simulink model "skarab_hmc_test"  (R2018a)
settings: Solver=VariableStepDiscrete  StartTime=0.0  StopTime=256.0  RelTol=1e-3
libraries: xbsIndex_r4 x424, xps_library x2
(part 1 of 4)
settings Model: Creator=omer  LastModifiedBy=hpw1
settings DataIOCC: LimitDataPoints=on  SaveFormat=Array
settings OptimizationCC: DefaultParameterBehavior=Inlined  ExpressionDepthLimit=2147483647  LifeSpan=inf
settings DebuggingCC: UnderspecifiedInitializationDetection=Classic  MergeDetectMultiDrivingBlocksExec=none  SolverPrmCheckMsg=warning  AllowSymbolicDim=off  StateNameClashWarn=warning  LibraryContextMissingDiagnostic=warning  SFUnexpectedBacktrackingDiag=warning  SFNoUnconditionalDefaultTransitionDiag=warning  SFExecutionAtInitializationDiag=none
settings HardwareCC: ProdBitPerPointer=32  ProdBitPerSizeT=32  ProdBitPerPtrDiffT=32  ProdLargestAtomicFloat=None  ProdIntDivRoundTo=Undefined  ProdEndianess=Unspecified  ProdWordSize=32  ProdHWDeviceType=32-bit Generic
settings ModelReferenceCC: PropagateSignalLabelsOutOfModel=off
settings CodeAppCC: StateflowObjectComments=on
settings GRTTargetCC: TargetLangStandard=C89/C90 (ANSI)  GeneratePreprocessorConditionals=Disable all
settings ConfigComp: CovMetricSettings=dw  CovHtmlReporting=on  CovSaveCumulativeToWorkspaceVar=on  CovSaveSingleToWorkspaceVar=on  CovExternalEMLEnable=off

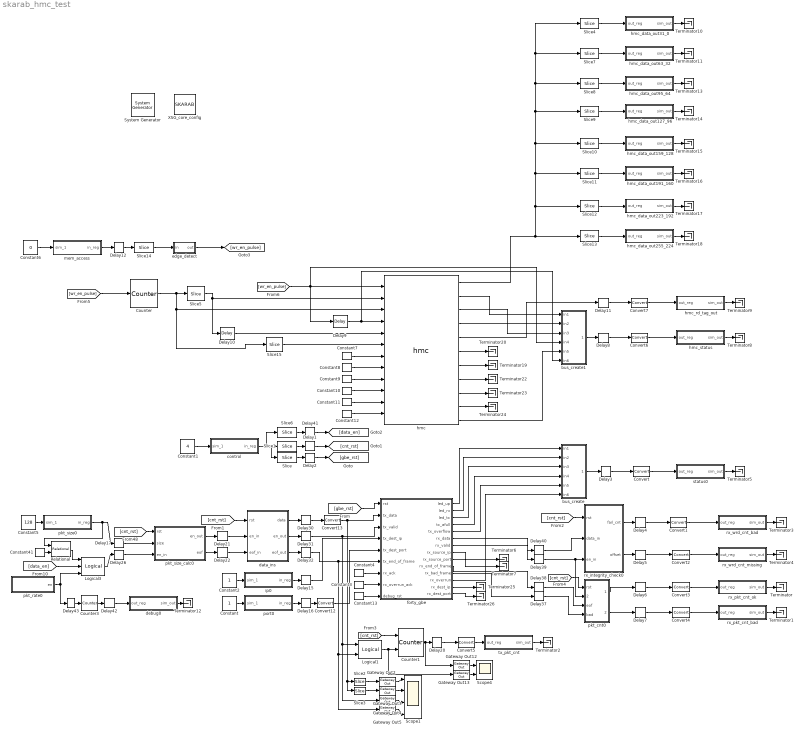
== system skarab_hmc_test ==
  " System Generator" : xbsIndex_r4/ System Generator  Tag=genX  xilinxfamily=virtex7  part=xc7vx690t  speed=-2  package=ffg1927  synthesis_tool=XST  clock_wrapper=Clock Enables  directory=/home/aisaacson/work/git_work/ska_sa/projects/mlib_devel/jasper_library/test_models/skarab_hmc_test/sysgen  proj_type=Vivado  Synth_file=Vivado Synthesis Defaults  Impl_file=Vivado Implementation Defaults  testbench=off  simulink_period=1  sysclk_period=4.4444  dcm_input_clock_period=10  incr_netlist=off  trim_vbits=Everywhere in SubSystem  dbl_ovrd=According to Block Masks  core_generation=According to Block Masks  run_coregen=off  deprecated_control=off  eval_field=0  block_type=sysgen
  Constant : Constant
  Constant1 : Constant  Value=4
  Constant10 : xbsIndex_r4/Constant  const=0  gui_display_data_type=Boolean  arith_type=Boolean  n_bits=16  bin_pt=14  preci_type=Single  exp_width=8  frac_width=24  explicit_period=on  period=1  equ=P=C  opselect=C  inp2=PCIN>>17  opr=+  inp1=P  carry=CIN  dbl_ovrd=off  block_type=constant
      settings: block_version=11.4
  Constant11 : xbsIndex_r4/Constant  const=0  gui_display_data_type=Fixed-point  arith_type=Unsigned  n_bits=27  bin_pt=0  preci_type=Single  exp_width=8  frac_width=24  explicit_period=on  period=1  equ=P=C  opselect=C  inp2=PCIN>>17  opr=+  inp1=P  carry=CIN  dbl_ovrd=off  block_type=constant
      settings: block_version=11.4
  Constant12 : xbsIndex_r4/Constant  const=0  gui_display_data_type=Fixed-point  arith_type=Signed (2's comp)  n_bits=9  bin_pt=0  preci_type=Single  exp_width=8  frac_width=24  explicit_period=on  period=1  equ=P=C  opselect=C  inp2=PCIN>>17  opr=+  inp1=P  carry=CIN  dbl_ovrd=off  block_type=constant
      settings: block_version=11.4
  Constant13 : xbsIndex_r4/Constant  const=0  gui_display_data_type=Boolean  arith_type=Boolean  n_bits=16  bin_pt=14  preci_type=Single  exp_width=8  frac_width=24  explicit_period=on  period=1  equ=P=C  opselect=C  inp2=PCIN>>17  opr=+  inp1=P  carry=CIN  dbl_ovrd=off  block_type=constant
      settings: block_version=11.4
  Constant2 : Constant
  Constant3 : xbsIndex_r4/Constant  const=1  gui_display_data_type=Fixed-point  arith_type=Boolean  n_bits=16  bin_pt=14  preci_type=Single  exp_width=8  frac_width=24  explicit_period=on  period=1  equ=P=C  opselect=C  inp2=PCIN>>17  opr=+  inp1=P  carry=CIN  dbl_ovrd=off  block_type=constant
      settings: block_version=11.4
  Constant4 : xbsIndex_r4/Constant  const=1  gui_display_data_type=Fixed-point  arith_type=Boolean  n_bits=16  bin_pt=14  preci_type=Single  exp_width=8  frac_width=24  explicit_period=on  period=1  equ=P=C  opselect=C  inp2=PCIN>>17  opr=+  inp1=P  carry=CIN  dbl_ovrd=off  block_type=constant
      settings: block_version=11.4
  Constant41 : xbsIndex_r4/Constant  const=0  gui_display_data_type=Fixed-point  arith_type=Unsigned  n_bits=32  bin_pt=0  preci_type=Single  exp_width=8  frac_width=24  explicit_period=on  period=1  equ=P=C  opselect=C  inp2=PCIN>>17  opr=+  inp1=P  carry=CIN  dbl_ovrd=off  block_type=constant
  Constant5 : Constant  Value=128
  Constant6 : Constant  Value=0
  Constant7 : xbsIndex_r4/Constant  const=0  gui_display_data_type=Boolean  arith_type=Boolean  n_bits=16  bin_pt=14  preci_type=Single  exp_width=8  frac_width=24  explicit_period=on  period=1  equ=P=C  opselect=C  inp2=PCIN>>17  opr=+  inp1=P  carry=CIN  dbl_ovrd=off  block_type=constant
      settings: block_version=11.4
  Constant8 : xbsIndex_r4/Constant  const=0  gui_display_data_type=Fixed-point  arith_type=Unsigned  n_bits=27  bin_pt=0  preci_type=Single  exp_width=8  frac_width=24  explicit_period=on  period=1  equ=P=C  opselect=C  inp2=PCIN>>17  opr=+  inp1=P  carry=CIN  dbl_ovrd=off  block_type=constant
      settings: block_version=11.4
  Constant9 : xbsIndex_r4/Constant  const=0  gui_display_data_type=Fixed-point  arith_type=Signed (2's comp)  n_bits=256  bin_pt=0  preci_type=Single  exp_width=8  frac_width=24  explicit_period=on  period=1  equ=P=C  opselect=C  inp2=PCIN>>17  opr=+  inp1=P  carry=CIN  dbl_ovrd=off  block_type=constant
      settings: block_version=11.4
  Convert{,1..7} (8 alike) : xbsIndex_r4/Convert  gui_display_data_type=Fixed-point  arith_type=Unsigned  n_bits=32  bin_pt=0  float_type=Single  exp_bits=8  fraction_bits=24  quantization=Truncate  overflow=Wrap  en=off  latency=0  pipeline=off  dbl_ovrd=off  block_type=convert
  Convert12 : xbsIndex_r4/Convert  gui_display_data_type=Fixed-point  arith_type=Unsigned  n_bits=16  bin_pt=0  float_type=Single  exp_bits=8  fraction_bits=24  quantization=Truncate  overflow=Wrap  en=off  latency=0  pipeline=off  dbl_ovrd=off  block_type=convert
  Convert13 : xbsIndex_r4/Convert  gui_display_data_type=Fixed-point  arith_type=Unsigned  n_bits=256  bin_pt=0  float_type=Single  exp_bits=8  fraction_bits=24  quantization=Truncate  overflow=Wrap  en=off  latency=0  pipeline=off  dbl_ovrd=off  block_type=convert
  Counter : xbsIndex_r4/Counter  cnt_type=Free Running  cnt_to=Inf  operation=Up  start_count=0  cnt_by_val=1  arith_type=Unsigned  n_bits=32  bin_pt=0  load_pin=off  rst=off  en=on  explicit_period=on  period=1  use_behavioral_HDL=off  implementation=Fabric  dbl_ovrd=off  block_type=counter
  Counter1 : xbsIndex_r4/Counter  cnt_type=Free Running  cnt_to=Inf  operation=Up  start_count=0  cnt_by_val=1  arith_type=Unsigned  n_bits=32  bin_pt=0  load_pin=off  rst=on  en=on  explicit_period=on  period=1  use_behavioral_HDL=off  implementation=Fabric  dbl_ovrd=off  block_type=counter
      settings: block_version=11.4
  Counter3 : xbsIndex_r4/Counter  cnt_type=Free Running  cnt_to=Inf  operation=Up  start_count=0  cnt_by_val=1  arith_type=Unsigned  n_bits=32  bin_pt=0  load_pin=off  rst=off  en=on  explicit_period=on  period=1  use_behavioral_HDL=off  implementation=Fabric  dbl_ovrd=off  block_type=counter
      settings: block_version=11.4
  Delay{1..8,11..12,15..17,20..22,26,30..32,37..43} (27 alike) : xbsIndex_r4/Delay  rst=off  infoeditControl=Selection of Reset will increase slice count due to use of real FFs and instead of SRLs  en=off  latency=1  reg_retiming=on  dbl_ovrd=off  block_type=delay
      settings: block_version=11.4
  Delay10 : xbsIndex_r4/Delay  rst=off  infoeditControl=Selection of Reset will increase slice count due to use of real FFs and instead of SRLs  en=off  latency=10  reg_retiming=off  dbl_ovrd=off  block_type=delay
  Delay9 : xbsIndex_r4/Delay  rst=off  infoeditControl=Selection of Reset will increase slice count due to use of real FFs and instead of SRLs  en=off  latency=10  reg_retiming=off  dbl_ovrd=off  block_type=delay
  Gateway Out{2..5,12..13} (6 alike) : xbsIndex_r4/Gateway Out  inherit_from_input=off  hdl_port=on  rows=1  columns=1  UseAsDAC=off  DACChannel='1'  interface=None  automatic_assignment=on  address_offset=hex2dec('00')  intf_name=''  intf_description=''  timing_constraint=None  locs_specified=off  LOCs={}  io_standard={}  block_type=gatewayout
      settings: infoedit="Gateway out block.  Converts Xilinx fixed point inputs into ouputs of type Simulink integer, double, or fixed point.<br><br>Hardware notes:  In hardware these blocks become top level output ports or are discarded, depending on how they are configured."  block_version=11.4
  Logical1 : xbsIndex_r4/Logical  logical_function=AND  inputs=2  en=off  latency=1  precision=Full  arith_type=Unsigned  n_bits=16  bin_pt=0  align_bp=on  dbl_ovrd=off  block_type=logical
      settings: block_version=11.4
  Logical3 : xbsIndex_r4/Logical  logical_function=AND  inputs=3  en=off  latency=1  precision=Full  arith_type=Unsigned  n_bits=16  bin_pt=0  align_bp=on  dbl_ovrd=off  block_type=logical
      settings: block_version=11.4
  Relational : xbsIndex_r4/Relational  mode=a>b  op_type=Bool  en=off  latency=2  dbl_ovrd=off  block_type=relational
  Scope1 : Scope  NumInputPorts=4
  Scope4 : Scope  NumInputPorts=2
  Slice : xbsIndex_r4/Slice  nbits=1  boolean_output=on  mode=Lower Bit Location + Width  bit1=0  base1=MSB of Input  bit0=0  base0=LSB of Input  dbl_ovrd=off  block_type=slice
  Slice1 : xbsIndex_r4/Slice  nbits=1  boolean_output=on  mode=Lower Bit Location + Width  bit1=0  base1=MSB of Input  bit0=1  base0=LSB of Input  dbl_ovrd=off  block_type=slice
  Slice10 : xbsIndex_r4/Slice  nbits=32  boolean_output=off  mode=Lower Bit Location + Width  bit1=0  base1=MSB of Input  bit0=128  base0=LSB of Input  dbl_ovrd=off  block_type=slice
  Slice11 : xbsIndex_r4/Slice  nbits=32  boolean_output=off  mode=Lower Bit Location + Width  bit1=0  base1=MSB of Input  bit0=160  base0=LSB of Input  dbl_ovrd=off  block_type=slice
  Slice12 : xbsIndex_r4/Slice  nbits=32  boolean_output=off  mode=Lower Bit Location + Width  bit1=0  base1=MSB of Input  bit0=192  base0=LSB of Input  dbl_ovrd=off  block_type=slice
  Slice13 : xbsIndex_r4/Slice  nbits=32  boolean_output=off  mode=Lower Bit Location + Width  bit1=0  base1=MSB of Input  bit0=224  base0=LSB of Input  dbl_ovrd=off  block_type=slice
  Slice14 : xbsIndex_r4/Slice  nbits=1  boolean_output=on  mode=Lower Bit Location + Width  bit1=0  base1=MSB of Input  bit0=0  base0=LSB of Input  dbl_ovrd=off  block_type=slice
  Slice15 : xbsIndex_r4/Slice  nbits=9  boolean_output=off  mode=Lower Bit Location + Width  bit1=0  base1=MSB of Input  bit0=0  base0=LSB of Input  dbl_ovrd=off  block_type=slice
  Slice2 : xbsIndex_r4/Slice  nbits=1  boolean_output=off  mode=Upper Bit Location + Width  bit1=0  base1=MSB of Input  bit0=1  base0=MSB of Input  dbl_ovrd=off  block_type=slice
  Slice3 : xbsIndex_r4/Slice  nbits=63  boolean_output=off  mode=Lower Bit Location + Width  bit1=0  base1=MSB of Input  bit0=0  base0=LSB of Input  dbl_ovrd=off  block_type=slice
  Slice4 : xbsIndex_r4/Slice  nbits=32  boolean_output=off  mode=Lower Bit Location + Width  bit1=0  base1=MSB of Input  bit0=0  base0=LSB of Input  dbl_ovrd=off  block_type=slice
  Slice5 : xbsIndex_r4/Slice  nbits=27  boolean_output=off  mode=Lower Bit Location + Width  bit1=0  base1=MSB of Input  bit0=0  base0=LSB of Input  dbl_ovrd=off  block_type=slice
  Slice6 : xbsIndex_r4/Slice  nbits=1  boolean_output=on  mode=Lower Bit Location + Width  bit1=0  base1=MSB of Input  bit0=2  base0=LSB of Input  dbl_ovrd=off  block_type=slice
  Slice7 : xbsIndex_r4/Slice  nbits=32  boolean_output=off  mode=Lower Bit Location + Width  bit1=0  base1=MSB of Input  bit0=32  base0=LSB of Input  dbl_ovrd=off  block_type=slice
  Slice8 : xbsIndex_r4/Slice  nbits=32  boolean_output=off  mode=Lower Bit Location + Width  bit1=0  base1=MSB of Input  bit0=64  base0=LSB of Input  dbl_ovrd=off  block_type=slice
  Slice9 : xbsIndex_r4/Slice  nbits=32  boolean_output=off  mode=Lower Bit Location + Width  bit1=0  base1=MSB of Input  bit0=96  base0=LSB of Input  dbl_ovrd=off  block_type=slice
  Terminator{,1..20,22..26} (26 alike) : Terminator
  XSG_core_config : xps_library/Platforms/SKARAB  Tag=xps:xsg  hw_sys=SKARAB:xc7vx690t  clk_src=sys_clk  clk_rate=225  sample_period=1  synthesis_tool=XST
      settings: SourceProductName=CASPER XPS Blockset
  bus_create : Subsystem  AncestorBlock=casper_library_flow_control/bus_create  mask(bus_create){inputNum=6}
      mask prompts: inputNum "Number of inputs:"
      mask init:
      | bus_create_init(gcb,...
      |     'inputNum', inputNum);
  bus_create1 : Subsystem  AncestorBlock=casper_library_flow_control/bus_create  mask(bus_create){inputNum=6}
      mask prompts: inputNum "Number of inputs:"
      mask init:
      | bus_create_init(gcb,...
      |     'inputNum', inputNum);
  control : Subsystem  Tag=xps:sw_reg  AncestorBlock=xps_library/Memory/software_register  mask(swreg){io_dir=From Processor, io_delay=0, init_val=0, sample_period=1, names=reg, bitwidths=32, bin_pts=0, arith_types=0, sim_port=on, show_format=on}
      mask prompts: io_dir "I/O direction"; io_delay "I/O delay"; init_val "Initial Value"; sample_period "Sample period"; names "Bitfield names [msb...lsb]"; bitwidths "Bitfield widths"; bin_pts "Bitfield binary pts"; arith_types "Bitfield types, ufix=0, fix=1, bool=2"; sim_port "Provide sim input/output?"; show_format "Print format string?"
      mask help: A 32-bit software-accessible register. Can be divided into bitfields of varying widths and types using the fields in the block mask.
      mask init:
      | swreg_init(gcb)
      settings: AttributesFormatString=1input:uf32.0 = 32 bits
      mask TypeOptions io_dir: To Processor | From Processor
      mask Callback io_dir:
      | mask_enables = get_param(gcb, 'MaskEnables');
      | mask_names = get_param(gcb, 'MaskNames');
      | if strcmp(get_param(gcb, 'io_dir'), 'To Processor'),
      |     mask_enables{ismember(mask_names, 'sample_period')} = 'off';
      | else
      |     mask_enables{ismember(mask_names, 'sample_period')} = 'on';
      | end
      | set_param(gcb, 'MaskEnables', mask_enables);
      mask DialogControl ParameterTabVar0 Prompt: Setup
  data_ins : Subsystem
  debug0 : Subsystem  Tag=xps:sw_reg  AncestorBlock=xps_library/Memory/software_register  mask(swreg){io_dir=To Processor, io_delay=0, init_val=0, sample_period=1, names=reg, bitwidths=32, bin_pts=0, arith_types=0, sim_port=on, show_format=on}
      mask prompts: io_dir "I/O direction"; io_delay "I/O delay"; init_val "Initial Value"; sample_period "Sample period"; names "Bitfield names [msb...lsb]"; bitwidths "Bitfield widths"; bin_pts "Bitfield binary pts"; arith_types "Bitfield types, ufix=0, fix=1, bool=2"; sim_port "Provide sim input/output?"; show_format "Print format string?"
      mask help: A 32-bit software-accessible register. Can be divided into bitfields of varying widths and types using the fields in the block mask.
      mask init:
      | swreg_init(gcb)
      settings: AttributesFormatString=1output:uf32.0 = 32 bits
      mask TypeOptions io_dir: To Processor | From Processor
      mask Callback io_dir:
      | mask_enables = get_param(gcb, 'MaskEnables');
      | mask_names = get_param(gcb, 'MaskNames');
      | if strcmp(get_param(gcb, 'io_dir'), 'To Processor'),
      |     mask_enables{ismember(mask_names, 'sample_period')} = 'off';
      | else
      |     mask_enables{ismember(mask_names, 'sample_period')} = 'on';
      | end
      | set_param(gcb, 'MaskEnables', mask_enables);
      mask DialogControl ParameterTabVar0 Prompt: Setup
  edge_detect : Subsystem  AncestorBlock=casper_library_misc/edge_detect  mask(edge_detect){edge=Rising, polarity=Active High, x_in=[0 0.08 0.08 0.16 0.16 0.24 0.24 0.32 0.32 0.4], y_in=[-1 -1  1  1  1  1  1  1  1  1], x_out=[0.6 0.68 0.68 0.76 0.76 0.84 0.84 0.92 0.92 1], y_out=[-1 -1  1  1 -1 -1 -1 -1 -1 -1]}
      mask prompts: edge "Edge Type"; polarity "Output Polarity"; x_in "Input X Positions"; y_in "Input Y Positions"; x_out "Output X Positions"; y_out "Output Y Positions"
      mask help: Output is active for one-cycle after each edge of the specified type (i.e. rising, falling or both).
      mask init:
      | edge_detect_init(gcb,...
      |     'edge',edge,...
      |     'polarity',polarity,...
      |     'x_in',x_in,...
      |     'x_out',x_out,...
      |     'y_in',y_in,...
      |     'y_out',y_out);
      | 
      | x_in_num=str2num(getfield(getfield(get_param(gcb,'UserData'),'parameters'),'x_in'));
      | x_out_num=str2num(getfield(getfield(get_param(gcb,'UserData'),'parameters'),'x_out'));
      | y_in_num=str2num(getfield(getfield(get_param(gcb,'UserData'),'parameters'),'y_in'));
      | y_out_num=str2num(getfield(getfield(get_param(gcb,'UserData'),'parameters'),'y_out'));
      settings: AttributesFormatString=|
      | rising edges
      | active high
      mask Help: Output is active for one-cycle after each edge of the specified type (i.e. rising, falling, or both).  Latency is zero.
      mask TypeOptions edge: Rising | Falling | Both
      mask TypeOptions polarity: Active High | Active Low
      mask Display:
      | plot(x_in_num,0.5+y_in_num*0.2);
      | plot(x_out_num,0.5+y_out_num*0.2);
  forty_gbe : Subsystem  Tag=xps:forty_gbe  AncestorBlock=xps_library/IO/forty_gbe  mask(forty_gbe){flavour=cx4, slot=1, port_r1=0, port_r2_cx4=0, port_r2_sfpp=0, port=0, rx_dist_ram=on, large_frames=off, input_pipeline_delay=3, show_param=off, pre_emph_r2=0.74, pre_emph=3, post_emph_r2=0.18, rxeqmix_r2=7, swing_r2=940, swing=800, fab_en=on, fab_mac=hex2dec('123456780000'), fab_ip=192*(2^24) + 168*(2^16) + 5*(2^8) + 20*(2^0), fab_udp=10000, fab_gate=1, cpu_rx_en=on, cpu_tx_en=on, ttl=hex2dec('FF'), promisc_mode=off, debug_ctr_width=16, debug_en_all=off, debug_dis_all=off, txctr=off, txerrctr=off, txerrctr_len=100, txofctr=off, txfullctr=off, txvldctr=off, txsnaplen=0 - no snap, rxctr=off, rxerrctr=off, rxerrctr_len=100, rxofctr=off, rxbadctr=off, rxvldctr=off, rxeofctr=off, rxsnaplen=0 - no snap, rxsrcip=on, rxdstip=on}
      mask prompts: flavour "Mezzanine card flavour"; slot "Card slot"; port_r1 "Port"; port_r2_cx4 "Port"; port_r2_sfpp "Port"; rx_dist_ram "Shallow RX Fifo (Beware overruns!)"; large_frames "Enable Large TX Frames (8k+512)"; input_pipeline_delay "Incoming pipeline delay"; show_param "---------------------- Show Implementation Parameters -----------------------------------------------------------------------------------"; pre_emph_r2 "Pre-emphasis (dB)"; pre_emph "Pre-emphasis"; post_emph_r2 "Post-emphasis (dB)"; rxeqmix_r2 "Receive equalisation"; swing_r2 "Driver Swing Control (mVppd)"; swing "Differential swing"; fab_en "Enable fabric on startup"; fab_mac "Fabric MAC Address"; fab_ip "Fabric IP Address"; fab_udp "Fabric UDP Port"; fab_gate "Fabric Gateway"; cpu_rx_en "Enable CPU RX"; cpu_tx_en "Enable CPU TX"; promisc_mode "Promiscuous mode"; debug_ctr_width "Debug counter width"; debug_en_all "Enable all counters (overrides individual settings)"; debug_dis_all "Disable all counters (overrides individual settings)"; txctr "TX - core_txctr"; txerrctr "TX packet length error - core_txerrctr"; txerrctr_len "-- expected TX packet length"; txofctr "TX overflow - core_txofctr"; txfullctr "TX full - core_txfullctr"; txvldctr "TX valid cycle - core_txvldctr"; txsnaplen "TX snapshot length"; rxctr "RX - core_rxctr"; rxerrctr "RX packet length error - core_rxerrctr"; rxerrctr_len "-- expected RX packet length"; rxofctr "RX overflow - core_rxofctr"; rxbadctr "RX bad - core_rxbadctr"; rxvldctr "RX valid cycle - core_rxvldctr"; rxeofctr "RX eof - core_rxeofctr"; rxsnaplen "RX snapshot length"; rxsrcip "RX snapshot - include source IPs"; rxdstip "RX snapshot - include destination IPs"
      mask help: This block sends and receives UDP frames (packets). It accepts a 64 bit wide data stream with user-determined frame breaks. The data stream is wrapped in a UDP frame for transmission. Incoming UDP packets are unwrapped and the data presented as a 64 bit wide stream.
      mask init:
      | temp = eval(get_param(gcb, 'debug_ctr_width'));
      | if temp <= 0,
      |     error('Debug counters cannot be <= zero.');
      | end
      | forty_gbe_mask(gcb)
      settings: AttributesFormatString=incoming_latency=3
      mask TypeOptions flavour: sfp+ | cx4
      mask Callback flavour: forty_gbe_callback
      mask TypeOptions slot: 0 | 1
      mask TypeOptions port_r1: 0 | 1 | 2 | 3
      mask TypeOptions port_r2_cx4: 0 | 1 | 2
      mask TypeOptions port_r2_sfpp: 0 | 1 | 2 | 3
      mask TypeOptions port: 0 | 1 | 2 | 3
      mask Callback show_param: forty_gbe_callback
      mask TypeOptions pre_emph_r2: 0.15 | 0.3 | 0.45 | 0.61 | 0.74 | 0.91 | 1.07 | 1.25 | 1.36 | 1.55 | 1.74 | 1.94 | 2.11 | 2.32 | 2.54 | 2.77
      mask TypeOptions pre_emph: 0 | 1 | 2 | 3
      mask TypeOptions post_emph_r2: 0.18 | 0.19 | 0.2 | 0.39 | 0.63 | 0.82 | 1.07 | 1.32 | 1.6 | 1.65 | 1.94 | 2.21 | 2.52 | 2.76 | 3.08 | 3.41 | 3.77 | 3.97 | 4.36 | 4.73 | 5.16 | 5.47 | 5.93 | 6.38 | 6.89
      mask TypeOptions rxeqmix_r2: 0 | 1 | 2 | 3 | 4 | 5 | 6 | 7
      mask TypeOptions swing_r2: 110 | 210 | 310 | 400 | 480 | 570 | 660 | 740 | 810 | 880 | 940 | 990 | 1040 | 1080 | 1110 | 1130
      mask TypeOptions swing: 400 | 500 | 600 | 700 | 800
      mask Callback debug_en_all:
      | if strcmp(get_param(gcb, 'debug_en_all'), 'on')
      |     set_param(gcb, 'debug_dis_all', 'off')
      | end
      mask Callback debug_dis_all:
      | if strcmp(get_param(gcb, 'debug_dis_all'), 'on')
      |     set_param(gcb, 'debug_en_all', 'off')
      | end
      mask Callback txerrctr:
      | blk = gcb;
      | mask_visibilities = get_param(blk, 'MaskVisibilities');
      | mask_names = get_param(blk, 'MaskNames');
      | if strcmp(get_param(blk, 'txerrctr'), 'on')
      |     mask_visibilities{ismember(mask_names, 'txerrctr_len')} = 'on';
      | else
      |     mask_visibilities{ismember(mask_names, 'txerrctr_len')} = 'off';
      | end
      | set_param(blk, 'MaskVisibilities', mask_visibilities);
      mask TypeOptions txsnaplen: 0 - no snap | 256 | 512 | 1024 | 2048 | 4096 | 8192 | 16384
      mask Callback rxerrctr:
      | blk = gcb;
      | mask_visibilities = get_param(blk, 'MaskVisibilities');
      | mask_names = get_param(blk, 'MaskNames');
      | if strcmp(get_param(blk, 'rxerrctr'), 'on')
      |     mask_visibilities{ismember(mask_names, 'rxerrctr_len')} = 'on';
      | else
      |     mask_visibilities{ismember(mask_names, 'rxerrctr_len')} = 'off';
      | end
      | set_param(blk, 'MaskVisibilities', mask_visibilities);
      mask TypeOptions rxsnaplen: 0 - no snap | 256 | 512 | 1024 | 2048 | 4096 | 8192 | 16384
      mask DialogControl ParameterTabVar0 Prompt: Core
      mask DialogControl ParameterTabVar01 Prompt: Debug counters
      mask DialogControl Control2 Prompt: -------------------------------------
      mask DialogControl Control2_copy Prompt: -------------------------------------
  hmc : xps_library/Memory/hmc  Tag=xps:hmc  mez=0  sim_depth=10  sim_latency=5  sim_rand=on
      settings: SourceProductName=CASPER XPS Blockset
  hmc_data_out127_96 : Subsystem  Tag=xps:sw_reg  AncestorBlock=xps_library/Memory/software_register  mask(swreg){io_dir=To Processor, io_delay=0, init_val=0, sample_period=1, names=reg, bitwidths=32, bin_pts=0, arith_types=0, sim_port=on, show_format=on}
      mask prompts: io_dir "I/O direction"; io_delay "I/O delay"; init_val "Initial Value"; sample_period "Sample period"; names "Bitfield names [msb...lsb]"; bitwidths "Bitfield widths"; bin_pts "Bitfield binary pts"; arith_types "Bitfield types, ufix=0, fix=1, bool=2"; sim_port "Provide sim input/output?"; show_format "Print format string?"
      mask help: A 32-bit software-accessible register. Can be divided into bitfields of varying widths and types using the fields in the block mask.
      mask init:
      | swreg_init(gcb)
      settings: AttributesFormatString=1output:uf32.0 = 32 bits
      mask TypeOptions io_dir: To Processor | From Processor
      mask Callback io_dir:
      | mask_enables = get_param(gcb, 'MaskEnables');
      | mask_names = get_param(gcb, 'MaskNames');
      | if strcmp(get_param(gcb, 'io_dir'), 'To Processor'),
      |     mask_enables{ismember(mask_names, 'sample_period')} = 'off';
      | else
      |     mask_enables{ismember(mask_names, 'sample_period')} = 'on';
      | end
      | set_param(gcb, 'MaskEnables', mask_enables);
      mask DialogControl ParameterTabVar0 Prompt: Setup
  hmc_data_out159_128 : Subsystem  Tag=xps:sw_reg  AncestorBlock=xps_library/Memory/software_register  mask(swreg){io_dir=To Processor, io_delay=0, init_val=0, sample_period=1, names=reg, bitwidths=32, bin_pts=0, arith_types=0, sim_port=on, show_format=on}
      mask prompts: io_dir "I/O direction"; io_delay "I/O delay"; init_val "Initial Value"; sample_period "Sample period"; names "Bitfield names [msb...lsb]"; bitwidths "Bitfield widths"; bin_pts "Bitfield binary pts"; arith_types "Bitfield types, ufix=0, fix=1, bool=2"; sim_port "Provide sim input/output?"; show_format "Print format string?"
      mask help: A 32-bit software-accessible register. Can be divided into bitfields of varying widths and types using the fields in the block mask.
      mask init:
      | swreg_init(gcb)
      settings: AttributesFormatString=1output:uf32.0 = 32 bits
      mask TypeOptions io_dir: To Processor | From Processor
      mask Callback io_dir:
      | mask_enables = get_param(gcb, 'MaskEnables');
      | mask_names = get_param(gcb, 'MaskNames');
      | if strcmp(get_param(gcb, 'io_dir'), 'To Processor'),
      |     mask_enables{ismember(mask_names, 'sample_period')} = 'off';
      | else
      |     mask_enables{ismember(mask_names, 'sample_period')} = 'on';
      | end
      | set_param(gcb, 'MaskEnables', mask_enables);
      mask DialogControl ParameterTabVar0 Prompt: Setup
  hmc_data_out191_160 : Subsystem  Tag=xps:sw_reg  AncestorBlock=xps_library/Memory/software_register  mask(swreg){io_dir=To Processor, io_delay=0, init_val=0, sample_period=1, names=reg, bitwidths=32, bin_pts=0, arith_types=0, sim_port=on, show_format=on}
      mask prompts: io_dir "I/O direction"; io_delay "I/O delay"; init_val "Initial Value"; sample_period "Sample period"; names "Bitfield names [msb...lsb]"; bitwidths "Bitfield widths"; bin_pts "Bitfield binary pts"; arith_types "Bitfield types, ufix=0, fix=1, bool=2"; sim_port "Provide sim input/output?"; show_format "Print format string?"
      mask help: A 32-bit software-accessible register. Can be divided into bitfields of varying widths and types using the fields in the block mask.
      mask init:
      | swreg_init(gcb)
      settings: AttributesFormatString=1output:uf32.0 = 32 bits
      mask TypeOptions io_dir: To Processor | From Processor
      mask Callback io_dir:
      | mask_enables = get_param(gcb, 'MaskEnables');
      | mask_names = get_param(gcb, 'MaskNames');
      | if strcmp(get_param(gcb, 'io_dir'), 'To Processor'),
      |     mask_enables{ismember(mask_names, 'sample_period')} = 'off';
      | else
      |     mask_enables{ismember(mask_names, 'sample_period')} = 'on';
      | end
      | set_param(gcb, 'MaskEnables', mask_enables);
      mask DialogControl ParameterTabVar0 Prompt: Setup
  hmc_data_out223_192 : Subsystem  Tag=xps:sw_reg  AncestorBlock=xps_library/Memory/software_register  mask(swreg){io_dir=To Processor, io_delay=0, init_val=0, sample_period=1, names=reg, bitwidths=32, bin_pts=0, arith_types=0, sim_port=on, show_format=on}
      mask prompts: io_dir "I/O direction"; io_delay "I/O delay"; init_val "Initial Value"; sample_period "Sample period"; names "Bitfield names [msb...lsb]"; bitwidths "Bitfield widths"; bin_pts "Bitfield binary pts"; arith_types "Bitfield types, ufix=0, fix=1, bool=2"; sim_port "Provide sim input/output?"; show_format "Print format string?"
      mask help: A 32-bit software-accessible register. Can be divided into bitfields of varying widths and types using the fields in the block mask.
      mask init:
      | swreg_init(gcb)
      settings: AttributesFormatString=1output:uf32.0 = 32 bits
      mask TypeOptions io_dir: To Processor | From Processor
      mask Callback io_dir:
      | mask_enables = get_param(gcb, 'MaskEnables');
      | mask_names = get_param(gcb, 'MaskNames');
      | if strcmp(get_param(gcb, 'io_dir'), 'To Processor'),
      |     mask_enables{ismember(mask_names, 'sample_period')} = 'off';
      | else
      |     mask_enables{ismember(mask_names, 'sample_period')} = 'on';
      | end
      | set_param(gcb, 'MaskEnables', mask_enables);
      mask DialogControl ParameterTabVar0 Prompt: Setup
  hmc_data_out255_224 : Subsystem  Tag=xps:sw_reg  AncestorBlock=xps_library/Memory/software_register  mask(swreg){io_dir=To Processor, io_delay=0, init_val=0, sample_period=1, names=reg, bitwidths=32, bin_pts=0, arith_types=0, sim_port=on, show_format=on}
      mask prompts: io_dir "I/O direction"; io_delay "I/O delay"; init_val "Initial Value"; sample_period "Sample period"; names "Bitfield names [msb...lsb]"; bitwidths "Bitfield widths"; bin_pts "Bitfield binary pts"; arith_types "Bitfield types, ufix=0, fix=1, bool=2"; sim_port "Provide sim input/output?"; show_format "Print format string?"
      mask help: A 32-bit software-accessible register. Can be divided into bitfields of varying widths and types using the fields in the block mask.
      mask init:
      | swreg_init(gcb)
      settings: AttributesFormatString=1output:uf32.0 = 32 bits
      mask TypeOptions io_dir: To Processor | From Processor
      mask Callback io_dir:
      | mask_enables = get_param(gcb, 'MaskEnables');
      | mask_names = get_param(gcb, 'MaskNames');
      | if strcmp(get_param(gcb, 'io_dir'), 'To Processor'),
      |     mask_enables{ismember(mask_names, 'sample_period')} = 'off';
      | else
      |     mask_enables{ismember(mask_names, 'sample_period')} = 'on';
      | end
      | set_param(gcb, 'MaskEnables', mask_enables);
      mask DialogControl ParameterTabVar0 Prompt: Setup
  hmc_data_out31_0 : Subsystem  Tag=xps:sw_reg  AncestorBlock=xps_library/Memory/software_register  mask(swreg){io_dir=To Processor, io_delay=0, init_val=0, sample_period=1, names=reg, bitwidths=32, bin_pts=0, arith_types=0, sim_port=on, show_format=on}
      mask prompts: io_dir "I/O direction"; io_delay "I/O delay"; init_val "Initial Value"; sample_period "Sample period"; names "Bitfield names [msb...lsb]"; bitwidths "Bitfield widths"; bin_pts "Bitfield binary pts"; arith_types "Bitfield types, ufix=0, fix=1, bool=2"; sim_port "Provide sim input/output?"; show_format "Print format string?"
      mask help: A 32-bit software-accessible register. Can be divided into bitfields of varying widths and types using the fields in the block mask.
      mask init:
      | swreg_init(gcb)
      settings: AttributesFormatString=1output:uf32.0 = 32 bits
      mask TypeOptions io_dir: To Processor | From Processor
      mask Callback io_dir:
      | mask_enables = get_param(gcb, 'MaskEnables');
      | mask_names = get_param(gcb, 'MaskNames');
      | if strcmp(get_param(gcb, 'io_dir'), 'To Processor'),
      |     mask_enables{ismember(mask_names, 'sample_period')} = 'off';
      | else
      |     mask_enables{ismember(mask_names, 'sample_period')} = 'on';
      | end
      | set_param(gcb, 'MaskEnables', mask_enables);
      mask DialogControl ParameterTabVar0 Prompt: Setup
  hmc_data_out63_32 : Subsystem  Tag=xps:sw_reg  AncestorBlock=xps_library/Memory/software_register  mask(swreg){io_dir=To Processor, io_delay=0, init_val=0, sample_period=1, names=reg, bitwidths=32, bin_pts=0, arith_types=0, sim_port=on, show_format=on}
      mask prompts: io_dir "I/O direction"; io_delay "I/O delay"; init_val "Initial Value"; sample_period "Sample period"; names "Bitfield names [msb...lsb]"; bitwidths "Bitfield widths"; bin_pts "Bitfield binary pts"; arith_types "Bitfield types, ufix=0, fix=1, bool=2"; sim_port "Provide sim input/output?"; show_format "Print format string?"
      mask help: A 32-bit software-accessible register. Can be divided into bitfields of varying widths and types using the fields in the block mask.
      mask init:
      | swreg_init(gcb)
      settings: AttributesFormatString=1output:uf32.0 = 32 bits
      mask TypeOptions io_dir: To Processor | From Processor
      mask Callback io_dir:
      | mask_enables = get_param(gcb, 'MaskEnables');
      | mask_names = get_param(gcb, 'MaskNames');
      | if strcmp(get_param(gcb, 'io_dir'), 'To Processor'),
      |     mask_enables{ismember(mask_names, 'sample_period')} = 'off';
      | else
      |     mask_enables{ismember(mask_names, 'sample_period')} = 'on';
      | end
      | set_param(gcb, 'MaskEnables', mask_enables);
      mask DialogControl ParameterTabVar0 Prompt: Setup
  hmc_data_out95_64 : Subsystem  Tag=xps:sw_reg  AncestorBlock=xps_library/Memory/software_register  mask(swreg){io_dir=To Processor, io_delay=0, init_val=0, sample_period=1, names=reg, bitwidths=32, bin_pts=0, arith_types=0, sim_port=on, show_format=on}
      mask prompts: io_dir "I/O direction"; io_delay "I/O delay"; init_val "Initial Value"; sample_period "Sample period"; names "Bitfield names [msb...lsb]"; bitwidths "Bitfield widths"; bin_pts "Bitfield binary pts"; arith_types "Bitfield types, ufix=0, fix=1, bool=2"; sim_port "Provide sim input/output?"; show_format "Print format string?"
      mask help: A 32-bit software-accessible register. Can be divided into bitfields of varying widths and types using the fields in the block mask.
      mask init:
      | swreg_init(gcb)
      settings: AttributesFormatString=1output:uf32.0 = 32 bits
      mask TypeOptions io_dir: To Processor | From Processor
      mask Callback io_dir:
      | mask_enables = get_param(gcb, 'MaskEnables');
      | mask_names = get_param(gcb, 'MaskNames');
      | if strcmp(get_param(gcb, 'io_dir'), 'To Processor'),
      |     mask_enables{ismember(mask_names, 'sample_period')} = 'off';
      | else
      |     mask_enables{ismember(mask_names, 'sample_period')} = 'on';
      | end
      | set_param(gcb, 'MaskEnables', mask_enables);
      mask DialogControl ParameterTabVar0 Prompt: Setup
  hmc_rd_tag_out : Subsystem  Tag=xps:sw_reg  AncestorBlock=xps_library/Memory/software_register  mask(swreg){io_dir=To Processor, io_delay=0, init_val=0, sample_period=1, names=reg, bitwidths=32, bin_pts=0, arith_types=0, sim_port=on, show_format=on}
      mask prompts: io_dir "I/O direction"; io_delay "I/O delay"; init_val "Initial Value"; sample_period "Sample period"; names "Bitfield names [msb...lsb]"; bitwidths "Bitfield widths"; bin_pts "Bitfield binary pts"; arith_types "Bitfield types, ufix=0, fix=1, bool=2"; sim_port "Provide sim input/output?"; show_format "Print format string?"
      mask help: A 32-bit software-accessible register. Can be divided into bitfields of varying widths and types using the fields in the block mask.
      mask init:
      | swreg_init(gcb)
      settings: AttributesFormatString=1output:uf32.0 = 32 bits
      mask TypeOptions io_dir: To Processor | From Processor
      mask Callback io_dir:
      | mask_enables = get_param(gcb, 'MaskEnables');
      | mask_names = get_param(gcb, 'MaskNames');
      | if strcmp(get_param(gcb, 'io_dir'), 'To Processor'),
      |     mask_enables{ismember(mask_names, 'sample_period')} = 'off';
      | else
      |     mask_enables{ismember(mask_names, 'sample_period')} = 'on';
      | end
      | set_param(gcb, 'MaskEnables', mask_enables);
      mask DialogControl ParameterTabVar0 Prompt: Setup
  hmc_status : Subsystem  Tag=xps:sw_reg  AncestorBlock=xps_library/Memory/software_register  mask(swreg){io_dir=To Processor, io_delay=0, init_val=0, sample_period=1, names=reg, bitwidths=32, bin_pts=0, arith_types=0, sim_port=on, show_format=on}
      mask prompts: io_dir "I/O direction"; io_delay "I/O delay"; init_val "Initial Value"; sample_period "Sample period"; names "Bitfield names [msb...lsb]"; bitwidths "Bitfield widths"; bin_pts "Bitfield binary pts"; arith_types "Bitfield types, ufix=0, fix=1, bool=2"; sim_port "Provide sim input/output?"; show_format "Print format string?"
      mask help: A 32-bit software-accessible register. Can be divided into bitfields of varying widths and types using the fields in the block mask.
      mask init:
      | swreg_init(gcb)
      settings: AttributesFormatString=1output:uf32.0 = 32 bits
      mask TypeOptions io_dir: To Processor | From Processor
      mask Callback io_dir:
      | mask_enables = get_param(gcb, 'MaskEnables');
      | mask_names = get_param(gcb, 'MaskNames');
      | if strcmp(get_param(gcb, 'io_dir'), 'To Processor'),
      |     mask_enables{ismember(mask_names, 'sample_period')} = 'off';
      | else
      |     mask_enables{ismember(mask_names, 'sample_period')} = 'on';
      | end
      | set_param(gcb, 'MaskEnables', mask_enables);
      mask DialogControl ParameterTabVar0 Prompt: Setup
  ip0 : Subsystem  Tag=xps:sw_reg  AncestorBlock=xps_library/Memory/software_register  mask(swreg){io_dir=From Processor, io_delay=0, init_val=0, sample_period=1, names=reg, bitwidths=32, bin_pts=0, arith_types=0, sim_port=on, show_format=on}
      mask prompts: io_dir "I/O direction"; io_delay "I/O delay"; init_val "Initial Value"; sample_period "Sample period"; names "Bitfield names [msb...lsb]"; bitwidths "Bitfield widths"; bin_pts "Bitfield binary pts"; arith_types "Bitfield types, ufix=0, fix=1, bool=2"; sim_port "Provide sim input/output?"; show_format "Print format string?"
      mask help: A 32-bit software-accessible register. Can be divided into bitfields of varying widths and types using the fields in the block mask.
      mask init:
      | swreg_init(gcb)
      settings: AttributesFormatString=1input:uf32.0 = 32 bits
      mask TypeOptions io_dir: To Processor | From Processor
      mask Callback io_dir:
      | mask_enables = get_param(gcb, 'MaskEnables');
      | mask_names = get_param(gcb, 'MaskNames');
      | if strcmp(get_param(gcb, 'io_dir'), 'To Processor'),
      |     mask_enables{ismember(mask_names, 'sample_period')} = 'off';
      | else
      |     mask_enables{ismember(mask_names, 'sample_period')} = 'on';
      | end
      | set_param(gcb, 'MaskEnables', mask_enables);
      mask DialogControl ParameterTabVar0 Prompt: Setup
  mem_access : Subsystem  Tag=xps:sw_reg  AncestorBlock=xps_library/Memory/software_register  mask(swreg){io_dir=From Processor, io_delay=0, init_val=0, sample_period=1, names=reg, bitwidths=32, bin_pts=0, arith_types=0, sim_port=on, show_format=on}
      mask prompts: io_dir "I/O direction"; io_delay "I/O delay"; init_val "Initial Value"; sample_period "Sample period"; names "Bitfield names [msb...lsb]"; bitwidths "Bitfield widths"; bin_pts "Bitfield binary pts"; arith_types "Bitfield types, ufix=0, fix=1, bool=2"; sim_port "Provide sim input/output?"; show_format "Print format string?"
      mask help: A 32-bit software-accessible register. Can be divided into bitfields of varying widths and types using the fields in the block mask.
      mask init:
      | swreg_init(gcb)
      settings: AttributesFormatString=1input:uf32.0 = 32 bits
      mask TypeOptions io_dir: To Processor | From Processor
      mask Callback io_dir:
      | mask_enables = get_param(gcb, 'MaskEnables');
      | mask_names = get_param(gcb, 'MaskNames');
      | if strcmp(get_param(gcb, 'io_dir'), 'To Processor'),
      |     mask_enables{ismember(mask_names, 'sample_period')} = 'off';
      | else
      |     mask_enables{ismember(mask_names, 'sample_period')} = 'on';
      | end
      | set_param(gcb, 'MaskEnables', mask_enables);
      mask DialogControl ParameterTabVar0 Prompt: Setup
  pkt_cnt0 : Subsystem
  pkt_rate0 : Subsystem
  pkt_size0 : Subsystem  Tag=xps:sw_reg  AncestorBlock=xps_library/Memory/software_register  mask(swreg){io_dir=From Processor, io_delay=0, init_val=0, sample_period=1, names=reg, bitwidths=32, bin_pts=0, arith_types=0, sim_port=on, show_format=on}
      mask prompts: io_dir "I/O direction"; io_delay "I/O delay"; init_val "Initial Value"; sample_period "Sample period"; names "Bitfield names [msb...lsb]"; bitwidths "Bitfield widths"; bin_pts "Bitfield binary pts"; arith_types "Bitfield types, ufix=0, fix=1, bool=2"; sim_port "Provide sim input/output?"; show_format "Print format string?"
      mask help: A 32-bit software-accessible register. Can be divided into bitfields of varying widths and types using the fields in the block mask.
      mask init:
      | swreg_init(gcb)
      settings: AttributesFormatString=1input:uf32.0 = 32 bits
      mask TypeOptions io_dir: To Processor | From Processor
      mask Callback io_dir:
      | mask_enables = get_param(gcb, 'MaskEnables');
      | mask_names = get_param(gcb, 'MaskNames');
      | if strcmp(get_param(gcb, 'io_dir'), 'To Processor'),
      |     mask_enables{ismember(mask_names, 'sample_period')} = 'off';
      | else
      |     mask_enables{ismember(mask_names, 'sample_period')} = 'on';
      | end
      | set_param(gcb, 'MaskEnables', mask_enables);
      mask DialogControl ParameterTabVar0 Prompt: Setup
  pkt_size_calc0 : Subsystem
  port0 : Subsystem  Tag=xps:sw_reg  AncestorBlock=xps_library/Memory/software_register  mask(swreg){io_dir=From Processor, io_delay=0, init_val=0, sample_period=1, names=reg, bitwidths=32, bin_pts=0, arith_types=0, sim_port=on, show_format=on}
      mask prompts: io_dir "I/O direction"; io_delay "I/O delay"; init_val "Initial Value"; sample_period "Sample period"; names "Bitfield names [msb...lsb]"; bitwidths "Bitfield widths"; bin_pts "Bitfield binary pts"; arith_types "Bitfield types, ufix=0, fix=1, bool=2"; sim_port "Provide sim input/output?"; show_format "Print format string?"
      mask help: A 32-bit software-accessible register. Can be divided into bitfields of varying widths and types using the fields in the block mask.
      mask init:
      | swreg_init(gcb)
      settings: AttributesFormatString=1input:uf32.0 = 32 bits
      mask TypeOptions io_dir: To Processor | From Processor
      mask Callback io_dir:
      | mask_enables = get_param(gcb, 'MaskEnables');
      | mask_names = get_param(gcb, 'MaskNames');
      | if strcmp(get_param(gcb, 'io_dir'), 'To Processor'),
      |     mask_enables{ismember(mask_names, 'sample_period')} = 'off';
      | else
      |     mask_enables{ismember(mask_names, 'sample_period')} = 'on';
      | end
      | set_param(gcb, 'MaskEnables', mask_enables);
      mask DialogControl ParameterTabVar0 Prompt: Setup
  rx_integrity_check0 : Subsystem
  rx_pkt_cnt_bad : Subsystem  Tag=xps:sw_reg  AncestorBlock=xps_library/Memory/software_register  mask(swreg){io_dir=To Processor, io_delay=0, init_val=0, sample_period=1, names=reg, bitwidths=32, bin_pts=0, arith_types=0, sim_port=on, show_format=on}
      mask prompts: io_dir "I/O direction"; io_delay "I/O delay"; init_val "Initial Value"; sample_period "Sample period"; names "Bitfield names [msb...lsb]"; bitwidths "Bitfield widths"; bin_pts "Bitfield binary pts"; arith_types "Bitfield types, ufix=0, fix=1, bool=2"; sim_port "Provide sim input/output?"; show_format "Print format string?"
      mask help: A 32-bit software-accessible register. Can be divided into bitfields of varying widths and types using the fields in the block mask.
      mask init:
      | swreg_init(gcb)
      settings: AttributesFormatString=1output:uf32.0 = 32 bits
      mask TypeOptions io_dir: To Processor | From Processor
      mask Callback io_dir:
      | mask_enables = get_param(gcb, 'MaskEnables');
      | mask_names = get_param(gcb, 'MaskNames');
      | if strcmp(get_param(gcb, 'io_dir'), 'To Processor'),
      |     mask_enables{ismember(mask_names, 'sample_period')} = 'off';
      | else
      |     mask_enables{ismember(mask_names, 'sample_period')} = 'on';
      | end
      | set_param(gcb, 'MaskEnables', mask_enables);
      mask DialogControl ParameterTabVar0 Prompt: Setup
  rx_pkt_cnt_ok : Subsystem  Tag=xps:sw_reg  AncestorBlock=xps_library/Memory/software_register  mask(swreg){io_dir=To Processor, io_delay=0, init_val=0, sample_period=1, names=reg, bitwidths=32, bin_pts=0, arith_types=0, sim_port=on, show_format=on}
      mask prompts: io_dir "I/O direction"; io_delay "I/O delay"; init_val "Initial Value"; sample_period "Sample period"; names "Bitfield names [msb...lsb]"; bitwidths "Bitfield widths"; bin_pts "Bitfield binary pts"; arith_types "Bitfield types, ufix=0, fix=1, bool=2"; sim_port "Provide sim input/output?"; show_format "Print format string?"
      mask help: A 32-bit software-accessible register. Can be divided into bitfields of varying widths and types using the fields in the block mask.
      mask init:
      | swreg_init(gcb)
      settings: AttributesFormatString=1output:uf32.0 = 32 bits
      mask TypeOptions io_dir: To Processor | From Processor
      mask Callback io_dir:
      | mask_enables = get_param(gcb, 'MaskEnables');
      | mask_names = get_param(gcb, 'MaskNames');
      | if strcmp(get_param(gcb, 'io_dir'), 'To Processor'),
      |     mask_enables{ismember(mask_names, 'sample_period')} = 'off';
      | else
      |     mask_enables{ismember(mask_names, 'sample_period')} = 'on';
      | end
      | set_param(gcb, 'MaskEnables', mask_enables);
      mask DialogControl ParameterTabVar0 Prompt: Setup
  rx_wrd_cnt_bad : Subsystem  Tag=xps:sw_reg  AncestorBlock=xps_library/Memory/software_register  mask(swreg){io_dir=To Processor, io_delay=0, init_val=0, sample_period=1, names=reg, bitwidths=32, bin_pts=0, arith_types=0, sim_port=on, show_format=on}
      mask prompts: io_dir "I/O direction"; io_delay "I/O delay"; init_val "Initial Value"; sample_period "Sample period"; names "Bitfield names [msb...lsb]"; bitwidths "Bitfield widths"; bin_pts "Bitfield binary pts"; arith_types "Bitfield types, ufix=0, fix=1, bool=2"; sim_port "Provide sim input/output?"; show_format "Print format string?"
      mask help: A 32-bit software-accessible register. Can be divided into bitfields of varying widths and types using the fields in the block mask.
      mask init:
      | swreg_init(gcb)
      settings: AttributesFormatString=1output:uf32.0 = 32 bits
      mask TypeOptions io_dir: To Processor | From Processor
      mask Callback io_dir:
      | mask_enables = get_param(gcb, 'MaskEnables');
      | mask_names = get_param(gcb, 'MaskNames');
      | if strcmp(get_param(gcb, 'io_dir'), 'To Processor'),
      |     mask_enables{ismember(mask_names, 'sample_period')} = 'off';
      | else
      |     mask_enables{ismember(mask_names, 'sample_period')} = 'on';
      | end
      | set_param(gcb, 'MaskEnables', mask_enables);
      mask DialogControl ParameterTabVar0 Prompt: Setup
  rx_wrd_cnt_missing : Subsystem  Tag=xps:sw_reg  AncestorBlock=xps_library/Memory/software_register  mask(swreg){io_dir=To Processor, io_delay=0, init_val=0, sample_period=1, names=reg, bitwidths=32, bin_pts=0, arith_types=0, sim_port=on, show_format=on}
      mask prompts: io_dir "I/O direction"; io_delay "I/O delay"; init_val "Initial Value"; sample_period "Sample period"; names "Bitfield names [msb...lsb]"; bitwidths "Bitfield widths"; bin_pts "Bitfield binary pts"; arith_types "Bitfield types, ufix=0, fix=1, bool=2"; sim_port "Provide sim input/output?"; show_format "Print format string?"
      mask help: A 32-bit software-accessible register. Can be divided into bitfields of varying widths and types using the fields in the block mask.
      mask init:
      | swreg_init(gcb)
      settings: AttributesFormatString=1output:uf32.0 = 32 bits
      mask TypeOptions io_dir: To Processor | From Processor
      mask Callback io_dir:
      | mask_enables = get_param(gcb, 'MaskEnables');
      | mask_names = get_param(gcb, 'MaskNames');
      | if strcmp(get_param(gcb, 'io_dir'), 'To Processor'),
      |     mask_enables{ismember(mask_names, 'sample_period')} = 'off';
      | else
      |     mask_enables{ismember(mask_names, 'sample_period')} = 'on';
      | end
      | set_param(gcb, 'MaskEnables', mask_enables);
      mask DialogControl ParameterTabVar0 Prompt: Setup
  status0 : Subsystem  Tag=xps:sw_reg  AncestorBlock=xps_library/Memory/software_register  mask(swreg){io_dir=To Processor, io_delay=0, init_val=0, sample_period=1, names=reg, bitwidths=32, bin_pts=0, arith_types=0, sim_port=on, show_format=on}
      mask prompts: io_dir "I/O direction"; io_delay "I/O delay"; init_val "Initial Value"; sample_period "Sample period"; names "Bitfield names [msb...lsb]"; bitwidths "Bitfield widths"; bin_pts "Bitfield binary pts"; arith_types "Bitfield types, ufix=0, fix=1, bool=2"; sim_port "Provide sim input/output?"; show_format "Print format string?"
      mask help: A 32-bit software-accessible register. Can be divided into bitfields of varying widths and types using the fields in the block mask.
      mask init:
      | swreg_init(gcb)
      settings: AttributesFormatString=1output:uf32.0 = 32 bits
      mask TypeOptions io_dir: To Processor | From Processor
      mask Callback io_dir:
      | mask_enables = get_param(gcb, 'MaskEnables');
      | mask_names = get_param(gcb, 'MaskNames');
      | if strcmp(get_param(gcb, 'io_dir'), 'To Processor'),
      |     mask_enables{ismember(mask_names, 'sample_period')} = 'off';
      | else
      |     mask_enables{ismember(mask_names, 'sample_period')} = 'on';
      | end
      | set_param(gcb, 'MaskEnables', mask_enables);
      mask DialogControl ParameterTabVar0 Prompt: Setup
  tx_pkt_cnt : Subsystem  Tag=xps:sw_reg  AncestorBlock=xps_library/Memory/software_register  mask(swreg){io_dir=To Processor, io_delay=0, init_val=0, sample_period=1, names=reg, bitwidths=32, bin_pts=0, arith_types=0, sim_port=on, show_format=on}
      mask prompts: io_dir "I/O direction"; io_delay "I/O delay"; init_val "Initial Value"; sample_period "Sample period"; names "Bitfield names [msb...lsb]"; bitwidths "Bitfield widths"; bin_pts "Bitfield binary pts"; arith_types "Bitfield types, ufix=0, fix=1, bool=2"; sim_port "Provide sim input/output?"; show_format "Print format string?"
      mask help: A 32-bit software-accessible register. Can be divided into bitfields of varying widths and types using the fields in the block mask.
      mask init:
      | swreg_init(gcb)
      settings: AttributesFormatString=1output:uf32.0 = 32 bits
      mask TypeOptions io_dir: To Processor | From Processor
      mask Callback io_dir:
      | mask_enables = get_param(gcb, 'MaskEnables');
      | mask_names = get_param(gcb, 'MaskNames');
      | if strcmp(get_param(gcb, 'io_dir'), 'To Processor'),
      |     mask_enables{ismember(mask_names, 'sample_period')} = 'off';
      | else
      |     mask_enables{ismember(mask_names, 'sample_period')} = 'on';
      | end
      | set_param(gcb, 'MaskEnables', mask_enables);
      mask DialogControl ParameterTabVar0 Prompt: Setup
  wires:
  [wr_en_pulse] -> hmc/1, bus_create1/4(in4), Delay9/1
  Delay9/1 -> bus_create1/6(in6), hmc/4
  Slice15/1 -> hmc/6
  Slice5/1 -> hmc/2, Delay10/1
  Delay10/1 -> hmc/5
  hmc/1 -> Slice4/1, Slice7/1, Slice8/1, Slice9/1, Slice10/1, Slice11/1, Slice12/1, Slice13/1
  data_ins/1(data) -> Delay30/1
  control/1(in_reg) -> Slice/1, Slice1/1, Slice6/1
  Constant/1 -> port0/1(sim_1)
  Constant1/1 -> control/1(sim_1)
  port0/1(in_reg) -> Delay16/1
  Constant2/1 -> ip0/1(sim_1)
  ip0/1(in_reg) -> Delay15/1
  Constant3/1 -> forty_gbe/8(rx_overrun_ack)
  Constant4/1 -> forty_gbe/7(rx_ack)
  Constant5/1 -> pkt_size0/1(sim_1)
  pkt_size0/1(in_reg) -> Delay17/1, Relational/1
  pkt_size_calc0/1(en_out) -> Delay21/1
  pkt_size_calc0/2(eof) -> Delay22/1
  data_ins/2(en_out) -> Delay31/1
  data_ins/3(eof_out) -> Delay32/1
  [gbe_rst] -> forty_gbe/1(rst)
  [cnt_rst] -> data_ins/1(rst)
  Slice/1 -> Delay2/1
  Slice1/1 -> Delay1/1
  Delay1/1 -> [cnt_rst]
  Delay2/1 -> [gbe_rst]
  Gateway Out2/1 -> Scope1/1
  Gateway Out3/1 -> Scope1/2
  Gateway Out4/1 -> Scope1/3
  Gateway Out5/1 -> Scope1/4
  Slice2/1 -> Gateway Out2/1
  Slice3/1 -> Gateway Out3/1
  [cnt_rst] -> rx_integrity_check0/1(rst)
  forty_gbe/7(rx_valid) -> Delay39/1
  forty_gbe/6(rx_data) -> Delay40/1
  pkt_cnt0/1(ok_cnt) -> Delay6/1
  pkt_cnt0/2(bad_cnt) -> Delay7/1
  rx_pkt_cnt_ok/1(sim_out) -> Terminator/1
  rx_pkt_cnt_bad/1(sim_out) -> Terminator1/1
  forty_gbe/10(rx_end_of_frame) -> Delay38/1
  forty_gbe/11(rx_bad_frame) -> Delay37/1
  tx_pkt_cnt/1(sim_out) -> Terminator2/1
  Logical1/1 -> Counter1/2, Gateway Out13/1
  Counter1/1 -> Delay20/1, Gateway Out12/1
  [cnt_rst] -> Counter1/1
  [cnt_rst] -> pkt_cnt0/1(rst)
  rx_wrd_cnt_bad/1(sim_out) -> Terminator3/1
  rx_wrd_cnt_missing/1(sim_out) -> Terminator4/1
  rx_integrity_check0/1(fail_cnt) -> Delay4/1
  rx_integrity_check0/2(offset) -> Delay5/1
  forty_gbe/1(led_up) -> bus_create/1(in1)
  forty_gbe/2(led_rx) -> bus_create/2(in2)
  forty_gbe/3(led_tx) -> bus_create/3(in3)
  forty_gbe/4(tx_afull) -> bus_create/4(in4)
  forty_gbe/5(tx_overflow) -> bus_create/5(in5)
  forty_gbe/12(rx_overrun) -> bus_create/6(in6)
  status0/1(sim_out) -> Terminator5/1
  bus_create/1(bus_out) -> Delay3/1
  Delay3/1 -> Convert/1
  Delay4/1 -> Convert1/1
  Delay5/1 -> Convert2/1
  Delay6/1 -> Convert3/1
  Delay7/1 -> Convert4/1
  Delay17/1 -> pkt_size_calc0/2(size)
  Delay20/1 -> Convert5/1
  Delay21/1 -> data_ins/2(en_in)
  Delay22/1 -> data_ins/3(eof_in)
  Delay26/1 -> pkt_size_calc0/3(en_in)
  Delay30/1 -> Convert13/1
  Delay31/1 -> forty_gbe/3(tx_valid), Logical1/1, Gateway Out4/1
  Delay32/1 -> forty_gbe/6(tx_end_of_frame), Gateway Out5/1, Logical1/2
  Delay37/1 -> pkt_cnt0/4(bad)
  Delay38/1 -> pkt_cnt0/3(eof)
  Delay39/1 -> pkt_cnt0/2(valid), rx_integrity_check0/3(en_in)
  Delay40/1 -> rx_integrity_check0/2(data_in)
  Slice6/1 -> Delay41/1
  Delay41/1 -> [data_en]
  pkt_rate0/1(en) -> Delay43/1, Logical3/3
  Logical3/1 -> Delay26/1
  [data_en] -> Logical3/2
  Gateway Out12/1 -> Scope4/1
  Gateway Out13/1 -> Scope4/2
  debug0/1(sim_out) -> Terminator12/1
  Counter3/1 -> Delay42/1
  Delay42/1 -> debug0/1(out_reg)
  Delay43/1 -> Counter3/1
  Constant41/1 -> Relational/2
  Relational/1 -> Logical3/1
  [cnt_rst] -> pkt_size_calc0/1(rst)
  Convert/1 -> status0/1(out_reg)
  Convert1/1 -> rx_wrd_cnt_bad/1(out_reg)
  Convert2/1 -> rx_wrd_cnt_missing/1(out_reg)
  Convert3/1 -> rx_pkt_cnt_ok/1(out_reg)
  Convert4/1 -> rx_pkt_cnt_bad/1(out_reg)
  Convert5/1 -> tx_pkt_cnt/1(out_reg)
  forty_gbe/8(rx_source_ip) -> Terminator6/1
  forty_gbe/9(rx_source_port) -> Terminator7/1
  hmc_status/1(sim_out) -> Terminator8/1
  bus_create1/1(bus_out) -> Delay8/1
  Delay8/1 -> Convert6/1
  Convert6/1 -> hmc_status/1(out_reg)
  hmc_rd_tag_out/1(sim_out) -> Terminator9/1
  Delay11/1 -> Convert7/1
  Convert7/1 -> hmc_rd_tag_out/1(out_reg)
  hmc_data_out31_0/1(sim_out) -> Terminator10/1
  Slice4/1 -> hmc_data_out31_0/1(out_reg)
  hmc_data_out63_32/1(sim_out) -> Terminator11/1
  Slice7/1 -> hmc_data_out63_32/1(out_reg)
  hmc_data_out95_64/1(sim_out) -> Terminator13/1
  Slice8/1 -> hmc_data_out95_64/1(out_reg)
  hmc_data_out127_96/1(sim_out) -> Terminator14/1
  Slice9/1 -> hmc_data_out127_96/1(out_reg)
  hmc_data_out159_128/1(sim_out) -> Terminator15/1
  Slice10/1 -> hmc_data_out159_128/1(out_reg)
  hmc_data_out191_160/1(sim_out) -> Terminator16/1
  Slice11/1 -> hmc_data_out191_160/1(out_reg)
  hmc_data_out223_192/1(sim_out) -> Terminator17/1
  Slice12/1 -> hmc_data_out223_192/1(out_reg)
  hmc_data_out255_224/1(sim_out) -> Terminator18/1
  Slice13/1 -> hmc_data_out255_224/1(out_reg)
  Constant6/1 -> mem_access/1(sim_1)
  edge_detect/1(out) -> [wr_en_pulse]
  mem_access/1(in_reg) -> Delay12/1
  Delay12/1 -> Slice14/1
  Slice14/1 -> edge_detect/1(in)
  Counter/1 -> hmc/3, Slice15/1, Slice5/1
  [wr_en_pulse] -> Counter/1
  hmc/2 -> bus_create1/1(in1)
  hmc/4 -> bus_create1/2(in2)
  hmc/11 -> bus_create1/5(in5)
  Delay15/1 -> forty_gbe/4(tx_dest_ip)
  Constant7/1 -> hmc/7
  Constant8/1 -> hmc/8
  Constant9/1 -> hmc/9
  Constant10/1 -> hmc/10
  Constant11/1 -> hmc/11
  Constant12/1 -> hmc/12
  hmc/6 -> Terminator20/1
  hmc/7 -> Terminator19/1
  hmc/8 -> Terminator22/1
  hmc/9 -> Terminator23/1
  hmc/10 -> Terminator24/1
  Constant13/1 -> forty_gbe/9(debug_rst)
  forty_gbe/13(rx_dest_ip) -> Terminator25/1
  forty_gbe/14(rx_dest_port) -> Terminator26/1
  hmc/5 -> Delay11/1
  hmc/3 -> bus_create1/3(in3)
  Delay16/1 -> Convert12/1
  Convert12/1 -> forty_gbe/5(tx_dest_port)
  Convert13/1 -> forty_gbe/2(tx_data), Slice2/1, Slice3/1
